simulink model "RM3"  (R2021a)
settings: Solver=ode4  StartTime=0  StopTime=400  FixedStep=0.1  MaxStep=0.1  RelTol=1e-3  EnableMultiTasking=on
undefined symbols (not defined in the file or in its folder): body, constraint, geometry, hydroData, pto
libraries: WECSim_Lib_Body_Elements x2, WECSim_Lib_Constraints x1, WECSim_Lib_Frames x1, WECSim_Lib_PTOs x1
settings Model: Creator=mlawson  LastModifiedBy=kmruehl
settings SolverCC: ZeroCrossControl=DisableAll  AlgebraicLoopSolver=LineSearch  AutoInsertRateTranBlk=on
settings DataIOCC: SaveFormat=Array  SaveOutput=off  SaveTime=off  ReturnWorkspaceOutputs=off
settings OptimizationCC: LifeSpan=inf  SimCompilerOptimization=on
settings DebuggingCC: UnderspecifiedInitializationDetection=Classic  MergeDetectMultiDrivingBlocksExec=none  SolverPrmCheckMsg=warning  AllowSymbolicDim=off  StateNameClashWarn=warning  SFUnexpectedBacktrackingDiag=warning  SFNoUnconditionalDefaultTransitionDiag=warning  SFExecutionAtInitializationDiag=none  SFMachineParentedDataDiag=warning  ArithmeticOperatorsInVariantConditions=warning
settings HardwareCC: ProdBitPerPointer=32  ProdBitPerSizeT=32  ProdBitPerPtrDiffT=32  ProdLargestAtomicFloat=None  ProdIntDivRoundTo=Undefined  ProdEndianess=Unspecified  ProdWordSize=32  ProdHWDeviceType=32-bit Generic
settings ModelReferenceCC: PropagateSignalLabelsOutOfModel=off
settings SFSimCC: SimUseLocalCustomCode=off  CustomCodeUndefinedFunction=UseInterfaceOnly
settings RTWCC: RTWUseLocalCustomCode=off
settings CodeAppCC: StateflowObjectComments=on
settings GRTTargetCC: TargetLangStandard=C89/C90 (ANSI)
settings ConfigComp: CovMetricSettings=dw  CovSaveCumulativeToWorkspaceVar=on  CovSaveSingleToWorkspaceVar=on  CovExternalEMLEnable=off  CovSFcnEnable=off
settings SimscapeCC: SimscapeNormalizeSystem=off
settings ConfigurationSet: Description=SimMechanics 2G
settings ExplorerConfigSet: InternalSimMechanicsExplorerSettings="<ExplorerConfiguration><canonicalview>default</canonicalview><TilePanel><TileInfo><Tiles Columns=\"1\" Count=\"1\" Rows=\"1\"><Column Left=\"2\" Weight=\"1\"/><Column Left=\"1335\"/><Row Top=\"2\" Weight=\"1\"/><Row Top=\"911\"/><Tile Height=\"1\" Width=\"1\" X=\"0\" Y=\"0\"/></Tiles></TileInfo><SceneInfo><SceneViewer><BGColor><R>0.60000002384185791</R><G>0.60000002384185791</G><B>0.60000002384185791</B></BGColor><Camera><Position><X>365.37645888990272</X><Y>-369.82486814446582</Y><Z>359.64809521743916</Z></Position><Center><X>-6.7351450971904585</X><Y>2.2867358426280204</Y><Z>-12.463508769654169</Z></Center><Up><X>-0.40824829046386307</X><Y>0.40824829046386307</Y><Z>0.81649658092772615</Z></Up><Left>-57.820127362122818</Left><Right>57.820127362122818</Right><Bottom>-38.308817187253304</Bottom><Top>38.308817187253304</Top></Camera></SceneViewer></SceneInfo></TilePanel></ExplorerConfiguration>"

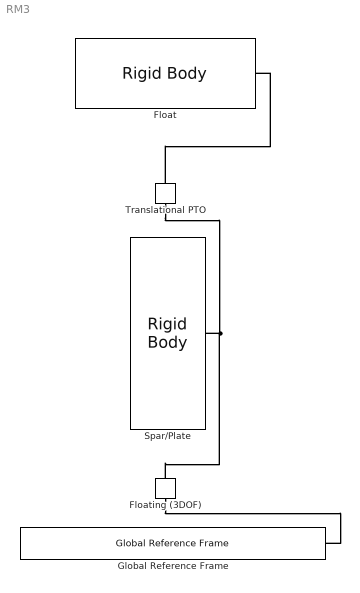
== system RM3 ==
  Float : WECSim_Lib_Body_Elements/Rigid Body  body=body(1)  h5File=hydroData/*.h5  geometryFile=geometry/*.stl  mass=0  inertia=0 0 0  nonHydro=0  nonlinearHydro=0  centerGravity=0 0 0  centerBuoyancy=0 0 0  dof=6  volume=0  displacement=0 0 0  axis=0 1 0  angle=0  option=0  cd=0 0 0  ca=0 0 0  area=0 0 0  VME=0  rgME=0 0 0  z=0 0 1
  Floating (3DOF) : WECSim_Lib_Constraints/Floating (3DOF)  constraint=constraint(1)  loc="0  0  0"  displacement=0 0 0  y=0 1 0  z=0 0 1  upperLimitSpecify=off  upperLimitBound=0  upperLimitTransitionRegionWidth=0  upperLimitStiffness=0  upperLimitDamping=0  lowerLimitSpecify=off  lowerLimitBound=0  lowerLimitTransitionRegionWidth=0  lowerLimitStiffness=0  lowerLimitDamping=0
      settings: AttributesFormatString=%<constraint>  SourceProductName=WEC-Sim
  Global Reference Frame : WECSim_Lib_Frames/Global Reference Frame  waves=waves  simu=simu  InputMethod=Input File  InputFile=wecSimInputFile.m  mode=normal  explorer=off  solver=ode4  startTime=0  rampTime=100  endTime=400  dt=0.1  cicEndTime=60  stateSpace=0  WaveClass=regular  height=2.5  period=8  elevationFile=NOT DEFINED  spectrumFile=NOT DEFINED  direction=0  spread=1  spectrumType=NOT DEFINED  phaseSeed=0  option=EqualEnergy
      settings: SourceProductName=WEC-Sim
  Spar/Plate : WECSim_Lib_Body_Elements/Rigid Body  body=body(2)  h5File=hydroData/*.h5  geometryFile=geometry/*.stl  mass=0  inertia=0 0 0  nonHydro=0  nonlinearHydro=0  centerGravity=0 0 0  centerBuoyancy=0 0 0  dof=6  volume=0  displacement=0 0 0  axis=0 1 0  angle=0  option=0  cd=0 0 0  ca=0 0 0  area=0 0 0  VME=0  rgME=0 0 0  z=0 0 1
  Translational PTO : WECSim_Lib_PTOs/Translational PTO  pto=pto(1)  loc="0  0  0"  stiffness=0  damping=0  equilibriumPosition=0  pretension=0  displacement=0 0 0  y=0 1 0  z=0 0 1  upperLimitSpecify=off  upperLimitBound=0  upperLimitTransitionRegionWidth=0  upperLimitStiffness=0  upperLimitDamping=0  lowerLimitSpecify=off  lowerLimitBound=0  lowerLimitTransitionRegionWidth=0  lowerLimitStiffness=0  lowerLimitDamping=0
      settings: AttributesFormatString=%<pto>  SourceProductName=WEC-Sim
  connections:
  Floating (3DOF)/LConn1 -- Global Reference Frame/RConn1
  Spar/Plate/RConn1 -- Floating (3DOF)/RConn1 -- Translational PTO/RConn1
  Translational PTO/LConn1 -- Float/RConn1
